simulink model "ex3"  (R2025b)
settings: Solver=VariableStepAuto  StartTime=0.0  StopTime=1  FixedStep=1e-4  RelTol=1e-4
values from neighbouring files (symbols this model uses):
  al = ap * 10    [sim3.m]
  Id_ref = psi_nominal_pu*psi_base/L_M    [sim3.m]
  Iq_ref = Te_nominal / ((3/2*K^2) * np * psi_nominal_pu*psi_base)    [sim3.m]
  ki = ac*(R_s+R_R+R_a)    [sim3.m]
  kip = ap*ap/psi_nominal    [sim3.m]
  kp = ac*L_sig    [sim3.m]
  kpp = 2*ap/psi_nominal    [sim3.m]
  L_sig = 0.0416    [sim3.m]
  R_a = ac*L_sig -(R_s+R_R)    [sim3.m]
  Te_nominal = Te_base * k    [sim3.m]
  V_base = sqrt(2) * K * (V_n)    [sim3.m]
settings Model: Creator=Dimitris  LastModifiedBy=Dimitris

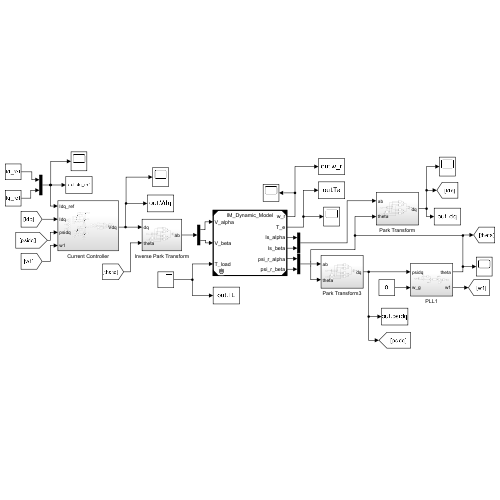
[thumbnail: Simulink's stored preview of the top-level diagram]
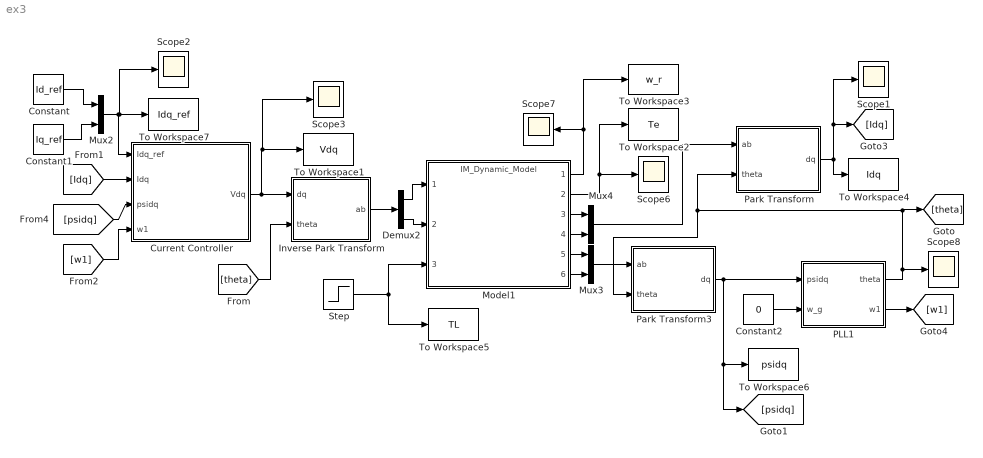
== system ex3 ==
  Constant : Constant  Value=Id_ref
  Constant1 : Constant  Value=Iq_ref
  Constant2 : Constant  Value=0
  Current Controller : Subsystem
  Demux2 : Demux  Outputs=2
  Inverse Park Transform : Subsystem
  Model1 : ModelReference  ModelNameDialog=IM_Dynamic_Model.slxp  ModelReferenceVersion=1.0  CopyOfModelProtected=on
  Mux2 : Mux  Inputs=2
  Mux3 : Mux  Inputs=2
  Mux4 : Mux  Inputs=2
  PLL1 : Subsystem
  Park Transform : Subsystem
  Park Transform3 : Subsystem
  Scope{1..3,6..8} (6 alike) : Scope
      Scope1 settings: ActiveDisplayYMinimum=-1.46523090740049  ActiveDisplayYMaximum=6.1362649288793731
      Scope2 settings: ActiveDisplayYMinimum=3.6592775926403838  ActiveDisplayYMaximum=5.2502678503101166  DataLoggingVariableName=ScopeData2
      Scope3 settings: ActiveDisplayYMinimum=-112.64302645002905  ActiveDisplayYMaximum=373.92551548520169  DataLoggingVariableName=ScopeData3
      Scope6 settings: ActiveDisplayYMinimum=-0.0029252213103024092  ActiveDisplayYMaximum=0.021242638855735789
      Scope7 settings: ActiveDisplayYMinimum=-98.616310603495748  ActiveDisplayYMaximum=480.65969750884744  DataLoggingVariableName=ScopeData6
      Scope8 settings: ActiveDisplayYMinimum=-0.78539816339744806  ActiveDisplayYMaximum=7.0685834705770345  DataLoggingVariableName=ScopeData7
  Step : Step  Time=0.5  After=Te_nominal*0.8  SampleTime=0
  To Workspace1 : ToWorkspace  VariableName=Vdq  SaveFormat=Timeseries  SampleTime=-1
  To Workspace2 : ToWorkspace  VariableName=Te  SaveFormat=Timeseries  SampleTime=-1
  To Workspace3 : ToWorkspace  VariableName=w_r  SaveFormat=Timeseries  SampleTime=-1
  To Workspace4 : ToWorkspace  VariableName=Idq  SaveFormat=Timeseries  SampleTime=-1
  To Workspace5 : ToWorkspace  VariableName=TL  SaveFormat=Timeseries  SampleTime=-1
  To Workspace6 : ToWorkspace  VariableName=psidq  SaveFormat=Timeseries  SampleTime=-1
  To Workspace7 : ToWorkspace  VariableName=Idq_ref  SaveFormat=Timeseries  SampleTime=-1
  wires:
  Current Controller/1(Vdq) -> Scope3/1, To Workspace1/1, Inverse Park Transform/1(dq)
  [Idq] -> Current Controller/2(Idq)
  Mux2/1 -> Scope2/1, To Workspace7/1, Current Controller/1(Idq_ref)
  Constant1/1 -> Mux2/2
  Constant/1 -> Mux2/1
  Inverse Park Transform/1(ab) -> Demux2/1
  PLL1/1(theta) -> Scope8/1, Park Transform3/2(theta), Park Transform/2(theta), [theta]
  Constant2/1 -> PLL1/2(w_g)
  Model1/4 -> Mux4/2
  Mux4/1 -> Park Transform/1(ab)
  Demux2/1 -> Model1/1
  Park Transform/1(dq) -> To Workspace4/1, [Idq], Scope1/1
  Step/1 -> To Workspace5/1, Model1/3
  Mux3/1 -> Park Transform3/1(ab)
  Demux2/2 -> Model1/2
  Model1/3 -> Mux4/1
  Model1/2 -> To Workspace2/1, Scope6/1
  Model1/6 -> Mux3/2
  Park Transform3/1(dq) -> [psidq], To Workspace6/1, PLL1/1(psidq)
  Model1/1 -> To Workspace3/1, Scope7/1
  Model1/5 -> Mux3/1
  [theta] -> Inverse Park Transform/2(theta)
  [psidq] -> Current Controller/3(psidq)
  [w1] -> Current Controller/4(w1)
  PLL1/2(w1) -> [w1]

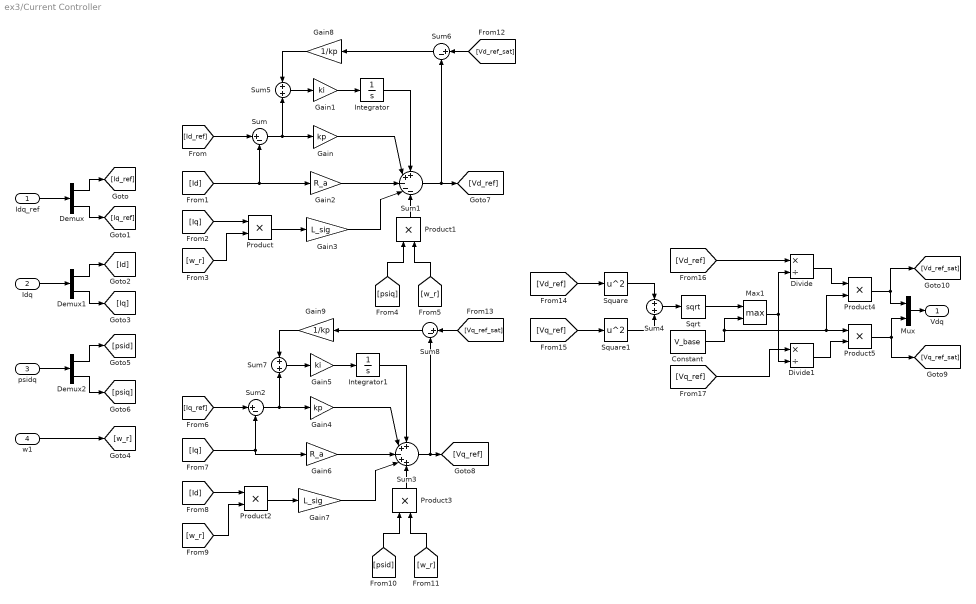
== system ex3/Current Controller ==
  Idq_ref : Inport
  Idq : Inport  Port=2
  psidq : Inport  Port=3
  w1 : Inport  Port=4
  Constant : Constant  Value=V_base
  Demux : Demux  Outputs=2
  Demux1 : Demux  Outputs=2
  Demux2 : Demux  Outputs=2
  Divide : Product  Inputs=*/
  Divide1 : Product  Inputs=*/
  Gain : Gain  Gain=kp
  Gain1 : Gain  Gain=ki
  Gain2 : Gain  Gain=R_a
  Gain3 : Gain  Gain=L_sig
  Gain4 : Gain  Gain=kp
  Gain5 : Gain  Gain=ki
  Gain6 : Gain  Gain=R_a
  Gain7 : Gain  Gain=L_sig
  Gain8 : Gain  Gain=1/kp
  Gain9 : Gain  Gain=1/kp
  Integrator : Integrator
  Integrator1 : Integrator
  Max1 : MinMax  Function=max  Inputs=2
  Mux : Mux  Inputs=2
  Product{,1..5} (6 alike) : Product
  Sqrt : Sqrt
  Square : Math  Operator=square
  Square1 : Math  Operator=square
  Sum{,2,6,8} (4 alike) : Sum  Inputs=|+-
  Sum1 : Sum  Inputs=++---
  Sum3 : Sum  Inputs=++-++
  Sum4 : Sum
  Sum5 : Sum
  Sum7 : Sum
  Vdq : Outport
  wires:
  Idq_ref/1 -> Demux/1
  Idq/1 -> Demux1/1
  Demux/1 -> [Id_ref]
  Demux/2 -> [Iq_ref]
  Demux1/1 -> [Id]
  Demux1/2 -> [Iq]
  [Id_ref] -> Sum/1
  [Id] -> Sum/2, Gain2/1
  Sum/1 -> Sum5/2, Gain/1
  Gain1/1 -> Integrator/1
  Integrator/1 -> Sum1/1
  Gain/1 -> Sum1/2
  Gain2/1 -> Sum1/3
  Gain3/1 -> Sum1/4
  Product/1 -> Gain3/1
  w1/1 -> [w_r]
  [Iq] -> Product/1
  [w_r] -> Product/2
  psidq/1 -> Demux2/1
  Demux2/1 -> [psid]
  Demux2/2 -> [psiq]
  [psiq] -> Product1/1
  [w_r] -> Product1/2
  Product1/1 -> Sum1/5
  Product3/1 -> Sum3/5
  [w_r] -> Product3/2
  [psid] -> Product3/1
  Product2/1 -> Gain7/1
  [Id] -> Product2/1
  Integrator1/1 -> Sum3/1
  Gain6/1 -> Sum3/3
  Gain5/1 -> Integrator1/1
  Gain7/1 -> Sum3/4
  Sum2/1 -> Sum7/2, Gain4/1
  [Iq_ref] -> Sum2/1
  [w_r] -> Product2/2
  [Iq] -> Gain6/1, Sum2/2
  Gain4/1 -> Sum3/2
  Sum1/1 -> [Vd_ref], Sum6/2
  [Vd_ref] -> Square/1
  [Vq_ref] -> Square1/1
  Square/1 -> Sum4/1
  Square1/1 -> Sum4/2
  Sum4/1 -> Sqrt/1
  Sqrt/1 -> Max1/1
  Max1/1 -> Divide/2, Divide1/2
  [Vd_ref] -> Divide/1
  [Vq_ref] -> Divide1/1
  Constant/1 -> Product4/2, Product5/1, Max1/2
  Mux/1 -> Vdq/1
  Sum5/1 -> Gain1/1
  Sum6/1 -> Gain8/1
  [Vd_ref_sat] -> Sum6/1
  Gain8/1 -> Sum5/1
  Sum7/1 -> Gain5/1
  Gain9/1 -> Sum7/1
  Sum3/1 -> Sum8/2, [Vq_ref]
  Sum8/1 -> Gain9/1
  [Vq_ref_sat] -> Sum8/1
  Divide/1 -> Product4/1
  Divide1/1 -> Product5/2
  Product5/1 -> [Vq_ref_sat], Mux/2
  Product4/1 -> [Vd_ref_sat], Mux/1

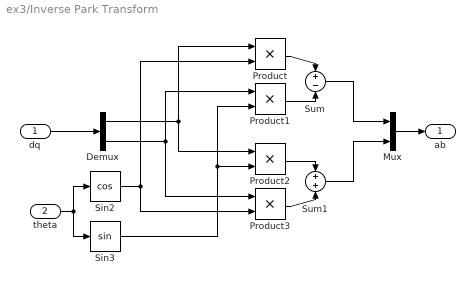
== system ex3/Inverse Park Transform ==
  dq : Inport
  theta : Inport  Port=2
  Demux : Demux  Outputs=2
  Mux : Mux  Inputs=2
  Product{,1..3} (4 alike) : Product
  Sin2 : Trigonometry  Operator=cos
  Sin3 : Trigonometry
  Sum : Sum  Inputs=+-
  Sum1 : Sum
  ab : Outport
  wires:
  Sum1/1 -> Mux/2
  Sin3/1 -> Product2/2, Product1/2
  Product1/1 -> Sum/2
  Demux/1 -> Product2/1, Product/1
  Mux/1 -> ab/1
  dq/1 -> Demux/1
  Sin2/1 -> Product/2, Product3/2
  Demux/2 -> Product1/1, Product3/1
  theta/1 -> Sin3/1, Sin2/1
  Sum/1 -> Mux/1
  Product/1 -> Sum/1
  Product3/1 -> Sum1/2
  Product2/1 -> Sum1/1

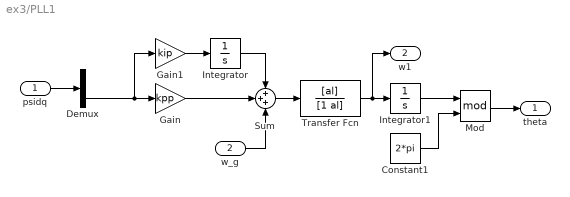
== system ex3/PLL1 ==
  psidq : Inport
  w_g : Inport  Port=2
  Constant1 : Constant  Value=2*pi
  Demux : Demux  Outputs=2
  Gain : Gain  Gain=kpp
  Gain1 : Gain  Gain=kip
  Integrator : Integrator
  Integrator1 : Integrator
  Mod : Math  Operator=mod
  Sum : Sum  Inputs=+++
  Transfer Fcn : TransferFcn  Numerator=[al]  Denominator=[1 al]
  theta : Outport
  w1 : Outport  Port=2
  wires:
  Gain1/1 -> Integrator/1
  Gain/1 -> Sum/2
  Sum/1 -> Transfer Fcn/1
  Transfer Fcn/1 -> w1/1, Integrator1/1
  Constant1/1 -> Mod/2
  Integrator1/1 -> Mod/1
  Mod/1 -> theta/1
  Demux/2 -> Gain1/1, Gain/1
  psidq/1 -> Demux/1
  Integrator/1 -> Sum/1
  w_g/1 -> Sum/3

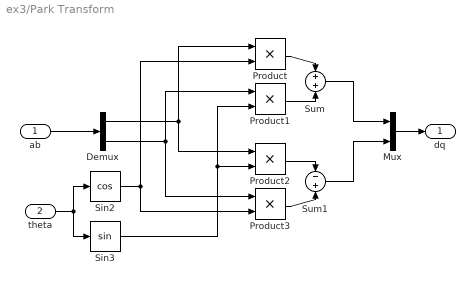
== system ex3/Park Transform ==
  ab : Inport
  theta : Inport  Port=2
  Demux : Demux  Outputs=2
  Mux : Mux  Inputs=2
  Product{,1..3} (4 alike) : Product
  Sin2 : Trigonometry  Operator=cos
  Sin3 : Trigonometry
  Sum : Sum
  Sum1 : Sum  Inputs=-+
  dq : Outport
  wires:
  Sin3/1 -> Product1/2, Product2/2
  Sin2/1 -> Product/2, Product3/2
  theta/1 -> Sin3/1, Sin2/1
  Demux/2 -> Product1/1, Product3/1
  Sum1/1 -> Mux/2
  Sum/1 -> Mux/1
  Demux/1 -> Product2/1, Product/1
  Product2/1 -> Sum1/1
  Product3/1 -> Sum1/2
  Product1/1 -> Sum/2
  Product/1 -> Sum/1
  Mux/1 -> dq/1
  ab/1 -> Demux/1

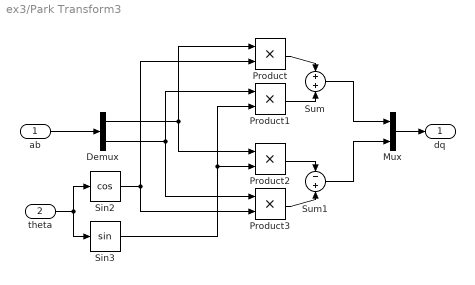
== system ex3/Park Transform3 ==
  ab : Inport
  theta : Inport  Port=2
  Demux : Demux  Outputs=2
  Mux : Mux  Inputs=2
  Product{,1..3} (4 alike) : Product
  Sin2 : Trigonometry  Operator=cos
  Sin3 : Trigonometry
  Sum : Sum
  Sum1 : Sum  Inputs=-+
  dq : Outport
  wires:
  Sin3/1 -> Product1/2, Product2/2
  Sin2/1 -> Product/2, Product3/2
  theta/1 -> Sin3/1, Sin2/1
  Demux/2 -> Product1/1, Product3/1
  Sum1/1 -> Mux/2
  Sum/1 -> Mux/1
  Demux/1 -> Product2/1, Product/1
  Product2/1 -> Sum1/1
  Product3/1 -> Sum1/2
  Product1/1 -> Sum/2
  Product/1 -> Sum/1
  Mux/1 -> dq/1
  ab/1 -> Demux/1
